simulink model "turbo_controller"  (R2025a)
settings: Solver=FixedStepAuto  StartTime=0.0  StopTime=inf  FixedStep=0.001  RelTol=1e-3
PostLoadFcn:
  | % 自动定位同目录CubeMX文件；不需要外部初始化脚本。
  | codertarget.data.setParameterValue('turbo_controller','STM32CubeMX.ProjectFile',fullfile(fileparts(get_param('turbo_controller','FileName')),'turbo_f407.ioc'));
InitFcn:
  | % 中文说明：按原控制器字段与类型创建三组接口总线；控制参数已内嵌。
  | tc_names=["EValve_Cycle" "EValve_Open" "Eblast_Cycle" "Eblast_Open" "Motor_Cycle" "Motor_Open" "EValve_Enable" "Eblast_Enable" "Motor_Enable" "SWO_Firework" "SWO_BleedAir" "EngineState" "Flag_ECUReset_Clear" "Flag_ECUReset_Save" "Flag_Reset_Enable" "Accelerator" "Nc_dem" "Nc"]; tc_types=["uint16" "uint16" "uint16" "uint16" "uint16" "uint16" "uint8" "uint8" "uint8" "uint8" "uint8" "uint8" "uint8" "uint8" "uint8" "single" "single" "single"];
  | for tc_k=1:numel(tc_names)
  |  tc_e(tc_k)=Simulink.BusElement; tc_e(tc_k).Name=char(tc_names(tc_k)); tc_e(tc_k).DataType=char(tc_types(tc_k));
  | end
  | EngineControl_Out=Simulink.Bus; EngineControl_Out.DataScope='Exported'; EngineControl_Out.Elements=tc_e;
  | clear tc_e tc_names tc_types tc_k
  | tc_names=["savedata1" "savedata2" "savedata3" "savedata4" "savedata5" "savedata6" "savedata7" "savedata8" "savedata9" "savedata10" "savedata11" "savedata12" "savedata13" "savedata14" "savedata15" "savedata16" "savedata17" "savedata18" "savedata19" "savedata20" "savedata21" "savedata22" "savedata23" "savedata24" "savedata25"]; tc_types=["single" "single" "single" "single" "single" "single" "single" "single" "single" "single" "single" "single" "single" "single" "single" "single" "single" "single" "single" "single" "single" "single" "single" "single" "single"];
  | for tc_k=1:numel(tc_names)
  |  tc_e(tc_k)=Simulink.BusElement; tc_e(tc_k).Name=char(tc_names(tc_k)); tc_e(tc_k).DataType=char(tc_types(tc_k));
  | end
  | SaveData_Out=Simulink.Bus; SaveData_Out.DataScope='Exported'; SaveData_Out.Elements=tc_e;
  | clear tc_e tc_names tc_types tc_k
  | tc_names=["senddata1" "senddata2" "senddata3" "senddata4" "senddata5" "senddata6" "senddata7" "senddata8" "senddata9" "senddata10" "senddata11" "senddata12" "senddata13" "senddata14" "senddata15" "senddata16" "senddata17" "senddata18" "senddata19" "senddata20" "senddata21" "senddata22" "senddata23" "senddata24" "senddata25" "senddata26" "senddata27" "senddata28" "senddata29"]; tc_types=["uint8" "uint8" "uint8" "uint8" "uint8" "uint8" "uint8" "uint8" "uint8" "uint8" "uint8" "uint8" "uint8" "uint8" "uint8" "uint8" "uint8" "uint8" "uint8" "uint8" "uint8" "uint8" "uint8" "uint8" "uint8" "uint8" "uint8" "uint8" "uint8"];
  | for tc_k=1:numel(tc_names)
  |  tc_e(tc_k)=Simulink.BusElement; tc_e(tc_k).Name=char(tc_names(tc_k)); tc_e(tc_k).DataType=char(tc_types(tc_k));
  | end
  | SendData_Out=Simulink.Bus; SendData_Out.DataScope='Exported'; SendData_Out.Elements=tc_e;
  | clear tc_e tc_names tc_types tc_k
  | 
  | % 以下为接口中文说明；只设置描述，不改变数值或数据类型。
  | EngineControl_Out.Description='执行控制输出（阀、电机、点火、状态及复位请求）';
  | tc_cn=["EValve_Cycle（主油阀周期计数（每计数2毫秒））" "EValve_Open（主油阀开通计数（每计数2毫秒））" "Eblast_Cycle（副油阀周期计数（每计数2毫秒））" "Eblast_Open（副油阀开通计数（每计数2毫秒））" "Motor_Cycle（起动电机周期计数）" "Motor_Open（起动电机开通计数）" "EValve_Enable（主油阀驱动使能）" "Eblast_Enable（副油阀驱动使能）" "Motor_Enable（起动电机使能）" "SWO_Firework（点火器使能（1开））" "SWO_BleedAir（引气阀使能（1开））" "EngineState（发动机状态）" "Flag_ECUReset_Clear（清除复位恢复状态请求）" "Flag_ECUReset_Save（保存复位恢复数据请求）" "Flag_Reset_Enable（处理器软件复位请求）" "Accelerator（油门／油泵给定控制量）" "Nc_dem（控制目标转速）" "Nc（发动机反馈转速（转每分））"];
  | tc_elements=EngineControl_Out.Elements;
  | for tc_k=1:numel(tc_cn)
  |  tc_elements(tc_k).Description=char(tc_cn(tc_k));
  | end
  | EngineControl_Out.Elements=tc_elements;
  | clear tc_cn tc_elements tc_k
  | SaveData_Out.Description='25项运行记录；字段含义按当前模型数据来源解释';
  | tc_cn=["savedata1（指令回显记录）" "savedata2（入口总温记录（℃））" "savedata3（电源电压记录）" "savedata4（排气温度记录（℃））" "savedata5（标定燃油压力记录）" "savedata6（副油阀占空比记录（％））" "savedata7（主油阀占空比记录（％））" "savedata8（温度修正转速记录）" "savedata9（开关输出及反馈位域）" "savedata10（物理转速记录）" "savedata11（油泵目标给定原始值）" "savedata12（起动电机占空比记录（％））" "savedata13（发动机状态码记录）" "savedata14（故障告警位域记录）" "savedata15（模型记录帧序号）" "savedata16（处理器温度记录（℃））" "savedata17（装订转速记录（沿用旧电源字段名））" "savedata18（导航高度记录）" "savedata19（飞行空速记录）" "savedata20（主阀旧记录位（恒零保留））" "savedata21（第21项保留记录（恒零））" "savedata22（保留记录项22）" "savedata23（保留记录项23）" "savedata24（保留记录项24）" "savedata25（保留记录项25）"];
  | tc_elements=SaveData_Out.Elements;
  | for tc_k=1:numel(tc_cn)
  |  tc_elements(tc_k).Description=char(tc_cn(tc_k));
  | end
  | SaveData_Out.Elements=tc_elements;
  | clear tc_cn tc_elements tc_k
  | SendData_Out.Description='29字段回传及外设命令接口；板端上位机帧只取第3至27字段';
  | tc_cn=["senddata1（回传发送允许标志（不直接上线路））" "senddata2（回传载荷长度25字节）" "senddata3（回传指令回显字节）" "senddata4（总温编码字节（℃＋80））" "senddata5（电源电压编码字节）" "senddata6（排温编码高字节）" "senddata7（排温编码低字节）" "senddata8（燃油压力编码高字节）" "senddata9（燃油压力编码低字节）" "senddata10（副油阀占空比字节（％））" "senddata11（主油阀占空比字节（％））" "senddata12（修正转速编码高字节）" "senddata13（修正转速编码低字节）" "senddata14（驱动及反馈状态位域）" "senddata15（物理转速编码高字节）" "senddata16（物理转速编码低字节）" "senddata17（油泵目标给定高字节（串口二使用））" "senddata18（油泵目标给定低字节（串口二使用））" "senddata19（起动电机占空比命令（串口一使用））" "senddata20（发动机状态码字节）" "senddata21（故障告警位域字节）" "senddata22（帧序号占位（板端另行填写））" "senddata23（处理器温度编码（℃＋50））" "senddata24（控制目标转速编码高字节）" "senddata25（控制目标转速编码低字节）" "senddata26（占位字节（板端改填实测泵速高字节））" "senddata27（占位字节（板端改填实测泵速低字节））" "senddata28（装订转速高字节（本板未发送））" "senddata29（装订转速低字节（本板未发送））"];
  | tc_elements=SendData_Out.Elements;
  | for tc_k=1:numel(tc_cn)
  |  tc_elements(tc_k).Description=char(tc_cn(tc_k));
  | end
  | SendData_Out.Elements=tc_elements;
  | clear tc_cn tc_elements tc_k
  | 
  | 
  | % FRAM模块化事务：接口类型和上电初始状态，随模型保存，无外部初始化文件。
  | clear FM_elements
  | FM_elements(1)=Simulink.BusElement;FM_elements(1).Name='phase';FM_elements(1).DataType='uint8';FM_elements(1).Dimensions=[1 1];FM_elements(1).Description='phase（当前事务阶段）';
  | FM_elements(2)=Simulink.BusElement;FM_elements(2).Name='a';FM_elements(2).DataType='uint8';FM_elements(2).Dimensions=[64 1];FM_elements(2).Description='a（启动时缓存的首区64字节）';
  | FM_elements(3)=Simulink.BusElement;FM_elements(3).Name='active';FM_elements(3).DataType='uint16';FM_elements(3).Dimensions=[1 1];FM_elements(3).Description='active（当前有效记录区地址）';
  | FM_elements(4)=Simulink.BusElement;FM_elements(4).Name='generation';FM_elements(4).DataType='uint32';FM_elements(4).Dimensions=[1 1];FM_elements(4).Description='generation（当前有效记录代号）';
  | FM_elements(5)=Simulink.BusElement;FM_elements(5).Name='record';FM_elements(5).DataType='uint8';FM_elements(5).Dimensions=[64 1];FM_elements(5).Description='record（本次冻结的待写记录）';
  | FM_elements(6)=Simulink.BusElement;FM_elements(6).Name='addr';FM_elements(6).DataType='uint16';FM_elements(6).Dimensions=[1 1];FM_elements(6).Description='addr（本次备用写入地址）';
  | FM_elements(7)=Simulink.BusElement;FM_elements(7).Name='lastSave';FM_elements(7).DataType='single';FM_elements(7).Dimensions=[1 1];FM_elements(7).Description='lastSave（上次开始保存的秒数）';
  | FM_elements(8)=Simulink.BusElement;FM_elements(8).Name='lastState';FM_elements(8).DataType='uint8';FM_elements(8).Dimensions=[1 1];FM_elements(8).Description='lastState（上次保存时的发动机状态）';
  | FM_elements(9)=Simulink.BusElement;FM_elements(9).Name='boot';FM_elements(9).DataType='boolean';FM_elements(9).Dimensions=[1 1];FM_elements(9).Description='boot（启动记录是否允许恢复）';
  | FM_elements(10)=Simulink.BusElement;FM_elements(10).Name='consumed';FM_elements(10).DataType='boolean';FM_elements(10).Dimensions=[1 1];FM_elements(10).Description='consumed（本次启动恢复通知是否已发送）';
  | FM_elements(11)=Simulink.BusElement;FM_elements(11).Name='payload';FM_elements(11).DataType='uint8';FM_elements(11).Dimensions=[20 1];FM_elements(11).Description='payload（当前20字节恢复内容）';
  | ... (+35 lines)
model workspace (MAT data in the model file):
  CRC16_Table_Reference = [0 4129 8258 12387 16516 20645 24774 28903 33032 37161 41290 45419 ... (256 elements, 256x1)]
  PE_Kaer = [0.15402 0.15402 0.12264 0.10076 0.09481 0.07601 0.07111 0.0569 0.05198 0.04926 0.05308 0.04325 ... (13 elements, 1x13)]
  PE_Nr = [21.2982 61.4260372 67.7475458 72.7394382 76.845934 80.6988798 83.8449282 86.6491912 88.9382406 89.178606 91.1938214 93.4068058 ... (13 elements, 1x13)]
  PE_Pump_Translate = 33.5999984741
  PE_RotaSpeed_Translate = 860
  PE_Taer = [0.4939154 0.4939154 0.40780982 0.34066978 0.31622756 0.30405716 0.34300244 0.26785022 0.37393554 0.23914836 0.44563948 0.31044662 ... (13 elements, 1x13)]
  PF_ACCFULLRANGE = 3360
  PF_Flag_ECUReset = 0
  PF_Flag_rx_suc = 1
  PF_Gear_Info = [40000; 45000; 50000; 55000; 57000; 59000; 60000; 61000; 61000; 61000; 61000; 61000]
  PF_K_TiaoJie = 1
  PF_Kpu = 10
  PF_MySet_Rxdata = [0 0 0 0 0 0 0 0 0 0 0 0 ... (50 elements, 50x1)]
  PF_MyUsart1_Rxdata = [0 0 0 0 0 0 0 0 0 0 0 0 ... (50 elements, 50x1)]
  PF_MyUsart2_Rxdata = [0 0 0 0 0 0 0 0 0 0 0 0 ... (50 elements, 50x1)]
  PF_Reset_Information = [0 0 0 0 0 0 0 0 0 0 0 0 ... (20 elements, 20x1)]
  PF_Sensor_X1_T4 = [0 4095]
  PF_Sensor_X2_T4 = [0 1.66666698456]
  PF_Sensor_X3_T4 = [0 504 999 1497 2010 2529 3051 3568 4076 4571 4959]
  PF_Sensor_X_P2 = [0.5 3]
  PF_Sensor_X_Poil = [0.5 3]
  PF_Sensor_X_T1t = [-50 300]
  PF_Sensor_X_Vpower = [0 3]
  PF_Sensor_X_Vpump = [0 3]
  PF_Sensor_Y1_T4 = [0 3]
  PF_Sensor_Y2_T4 = [0 5000]
  PF_Sensor_Y3_T4 = [0 100 200 300 400 500 600 700 800 900 980]
  PF_Sensor_Y_P2 = [0 1000]
  PF_Sensor_Y_Poil = [0 1000]
  PF_Sensor_Y_T1t = [-50 300]
  PF_Sensor_Y_Vpower = [0 33]
  PF_Sensor_Y_Vpump = [0 33]
  PG_CtrlMode_CloseLoop : mpt.Parameter (value not decoded)
  PG_CtrlMode_ManualAcc : mpt.Parameter (value not decoded)
  PG_CtrlMode_Origin : mpt.Parameter (value not decoded)
  PG_CtrlMode_Start : mpt.Parameter (value not decoded)
  PG_CtrlMode_Stop : mpt.Parameter (value not decoded)
  PG_ES_Clp : mpt.Parameter (value not decoded)
  PG_ES_EngStart : mpt.Parameter (value not decoded)
  PG_ES_Manual : mpt.Parameter (value not decoded)
  PG_ES_Origin : mpt.Parameter (value not decoded)
  PG_ES_Stop : mpt.Parameter (value not decoded)
  PG_Instr_BleedAirSet : mpt.Parameter (value not decoded)
  PG_Instr_CloseLoop : mpt.Parameter (value not decoded)
  PG_Instr_ECUReSet : mpt.Parameter (value not decoded)
  PG_Instr_EValveSet : mpt.Parameter (value not decoded)
  PG_Instr_EblastSet : mpt.Parameter (value not decoded)
  PG_Instr_Erase : mpt.Parameter (value not decoded)
  PG_Instr_FireWorkSet : mpt.Parameter (value not decoded)
  PG_Instr_ManualPlus : mpt.Parameter (value not decoded)
  PG_Instr_ManualrReduce : mpt.Parameter (value not decoded)
  PG_Instr_MotorSet : mpt.Parameter (value not decoded)
  PG_Instr_OilSet : mpt.Parameter (value not decoded)
  PG_Instr_SelfCheck : mpt.Parameter (value not decoded)
  PG_Instr_Start : mpt.Parameter (value not decoded)
  PG_Instr_Stop : mpt.Parameter (value not decoded)
  PG_Instr_StopZero : Simulink.Parameter (value not decoded)
  PG_Location_Air : Simulink.Parameter (value not decoded)
  PG_Location_Gnd : Simulink.Parameter (value not decoded)
  PG_ServoCtrlMode_CloseLoop : Simulink.Parameter (value not decoded)
  PG_ServoCtrlMode_CloseLoopMax : Simulink.Parameter (value not decoded)
  PG_ServoCtrlMode_CloseLoopMin : Simulink.Parameter (value not decoded)
  PG_ServoCtrlMode_ManualAcc : Simulink.Parameter (value not decoded)
  PG_ServoCtrlMode_ManualAccMax : Simulink.Parameter (value not decoded)
  PG_ServoCtrlMode_ManualAccMin : Simulink.Parameter (value not decoded)
  PG_SpeedDot_Permit : Simulink.Parameter (value not decoded)
  PL_EngineModel_Actuator = [0 10 100]
  PL_EngineModel_EngineStar_Press_P2 = [1013 1098.4 1099.144828 1099.931034 1103.613793 1162.662069 1143.793103 1131.006897 1123.186207 1117.6 1114 1111.806897 ... (127 elements, 1x127)]
  PL_EngineModel_EngineStar_RotaSpeed = [200 2000 9584 9660 10220 10240 10260 10288 10308 10368 10380 10408 ... (127 elements, 1x127)]
  PL_EngineModel_EngineStar_Temp_Exhaust = [128 129 129.1 130 131 131.1 132 133 134 134.1 135 135.1 ... (127 elements, 1x127)]
  PL_EngineModel_EngineStar_Time = [0.05 0.1 0.15 0.2 0.25 0.3 0.35 0.4 0.45 0.5 0.55 0.6 ... (127 elements, 1x127)]
  PL_EngineModel_IdleAbove_Nr = [0 21.2982 61.4260372 67.7475458 72.7394382 76.845934 80.6988798 83.8449282 86.6491912 88.9382406 89.178606 91.1938214 ... (14 elements, 1x14)]
  PL_EngineModel_IdleAbove_P2r = [0.986923266716 1.57907722675 1.81593881076 1.99358499877 2.23044658278 2.43770046879 2.65482358747 2.84233900814 3.03972366149 3.18776215149 3.25684678016 3.3950160375 ... (14 elements, 1x14)]
  PL_EngineModel_IdleAbove_Tempr = [0.0536001429337 1.07200285867 1.63301768805 1.63659103091 1.66875111667 1.72592460247 1.77595140254 1.86171163123 1.95461854565 2.03323208862 2.03323208862 2.13685903162 ... (14 elements, 1x14)]
  PL_EngineModel_IdleAbove_Ter = [0.42434128 0.42434128 0.42434128 0.30669408 0.23570008 0.22150128 0.1997974 0.23803274 0.16115638 0.24279948 0.13600422 0.31308354 ... (14 elements, 1x14)]
  PL_EngineModel_IdleAbove_Wfr = [0 10.142 23.8337 27.8905 31.9473 36.0041 40.0609 44.1177 48.1745 52.2313 52.7384 56.7952 ... (14 elements, 1x14)]
  PL_EngineModel_Press_P2 = [400 400 400 400 400 400 400 400 400 400]
  PL_EngineModel_Rotaspeed = [0 20000 96400]
  PL_EngineModel_Temp_Exhaust = [500 500 500 500 500 500 500 500 500 500]
  PL_Kaer = [0.1 0.1 0.1 0.1 0.1 0.1]
  PL_Nr = [50 60 70 80 90 100]
  PL_Taer = [0.1 0.1 0.1 0.1 0.1 0.1]
  Sig : Simulink.Signal (value not decoded)
  Ts_ms : Simulink.Parameter (value not decoded)
  false : Simulink.Parameter (value not decoded)
  true : Simulink.Parameter (value not decoded)
symbols that are objects in the model workspace (value not decoded): PG_CtrlMode_CloseLoop, PG_CtrlMode_ManualAcc, PG_CtrlMode_Origin, PG_CtrlMode_Start, PG_CtrlMode_Stop, PG_ES_Clp, PG_ES_EngStart, PG_ES_Manual, PG_ES_Origin, PG_ES_Stop, PG_Instr_BleedAirSet, PG_Instr_CloseLoop, PG_Instr_EblastSet, PG_Instr_ECUReSet, PG_Instr_Erase, PG_Instr_EValveSet, PG_Instr_FireWorkSet, PG_Instr_ManualPlus, PG_Instr_ManualrReduce, PG_Instr_MotorSet, PG_Instr_OilSet, PG_Instr_SelfCheck, PG_Instr_Start, PG_Instr_Stop, PG_Instr_StopZero, PG_ServoCtrlMode_CloseLoop, PG_ServoCtrlMode_CloseLoopMax, PG_ServoCtrlMode_CloseLoopMin, PG_ServoCtrlMode_ManualAcc, PG_ServoCtrlMode_ManualAccMax, PG_ServoCtrlMode_ManualAccMin, Ts_ms
libraries: simulink x97, stm32blockslib x10, stm32f4xxblockslib x8
(part 8 of 26)

== system turbo_controller/BoardOutput_串口封装与阀门时序/Out04_Command（电机及油泵指令） ==
  note: 给电机和油泵各生成一帧控制命令
      |
      | 这里使用上层执行控制和回传字段，按20 ms节拍生成两路外设命令，而不是解析外设回包。两路协议
      | 均为9字节：
      | AA 55 03 00 02 命令高字节 命令低字节 CRC高字节 CRC低字节。
      |
      | 电机这一路把命令高字节固定为0，低字节采用原电机给定。油泵这一路采用原有油泵给定的高低两个
      | 字节；不能把两路的字节来源互换。
      | MotorFrame和PumpFrame各自只对两个命令字节计算CRC，不把前五项固定头部加入校验。
      |
      | 到20 ms更新且相应发送条件成立时，输出帧和有效长度交Out05_Handoff，再送根层USART1/USART2发
      | 送模块。数据值为0也可能是一条有意义的停机命令，因此发送许可和命令是否为0是不同判断。
  Send（外设命令总线）_867 : Inport  OutDataTypeStr=Bus: SendData_Out
  Seconds（当前秒数）_868 : Inport  Port=2  OutDataTypeStr=double
  Commands（原油泵与电机给定字节）_876 : BusSelector  OutputSignals=senddata17,senddata18,senddata19
  Constant（常量）_869 : Constant  Value=1000  OutDataTypeStr=double
  Constant（常量）_872 : Constant  Value=20  OutDataTypeStr=double
  Constant（常量）_874 : Constant  Value=0  OutDataTypeStr=double
  Constant（常量）_924 : Constant  Value=0  OutDataTypeStr=uint8
  Constant（常量）_975 : Constant  Value=9  OutDataTypeStr=uint16
  Constant（常量）_976 : Constant  Value=0  OutDataTypeStr=uint16
  Every20ms（20毫秒更新许可）_875 : RelationalOperator  Operator===  OutDataTypeStr=boolean  RndMeth=Simplest  InputSameDT=off
  Format（保持原输出维度）_2 : Reshape
  Format（保持原输出维度）_4 : Reshape
  Length（二十毫秒发送九字节）_977 : Switch  Criteria=u2 ~= 0  SaturateOnIntegerOverflow=off  InputSameDT=off
  Milliseconds（秒换算为毫秒）_870 : Product  Inputs=**  SaturateOnIntegerOverflow=on  OutDataTypeStr=Inherit: Same as first input
  MotorFrame（电机指令高字节固定为零）_925 : Subsystem  Description=|
      | 电机的两个命令字节怎样装成九字节帧
      | 
      | 父级把高命令字节固定0，低命令字节来自电机给定。这里不重新决定给定大小，只把这两个字节包装为外设协议。
      | 
      | 前五项固定为十六进制AA、55、03、00、02；第6、7项依次放命令高字节与低字节。CRC16只以第6、7两项为输入，计算出16位校验值，再把CRC高字节放第8项、低字节放第9项。
      | 
      | 完整帧 = [AA;55;03;00;02;CmdH;CmdL;CRCH;CRCL]。
      | 例如命令高0、低100表示两字节数100；CRC必须用[0,100]按本工程CRC表算出，不能只校验100或把AA55头部也算进去。
      | 
      | 9项帧交给父级，由20 ms发送许可和长度控制是否实际发送；本模块本身不操作串口。
  NoFrame（非通信毫秒输出零帧）_974 : Constant  Value=zeros(9,1)  OutDataTypeStr=uint8
  Phase20（20毫秒相位）_873 : Math  Operator=mod
  PumpFrame（油泵指令使用原高低给定字节）_973 : Subsystem  Description=|
      | 油泵的两个命令字节怎样装成九字节帧
      | 
      | 父级传入原油泵给定的高、低两个命令字节。这里不重新决定给定大小，只把这两个字节包装为外设协议。
      | 
      | 前五项固定为十六进制AA、55、03、00、02；第6、7项依次放命令高字节与低字节。CRC16只以第6、7两项为输入，计算出16位校验值，再把CRC高字节放第8项、低字节放第9项。
      | 
      | 完整帧 = [AA;55;03;00;02;CmdH;CmdL;CRCH;CRCL]。
      | 例如命令高0、低100表示两字节数100；CRC必须用[0,100]按本工程CRC表算出，不能只校验100或把AA55头部也算进去。
      | 
      | 9项帧交给父级，由20 ms发送许可和长度控制是否实际发送；本模块本身不操作串口。
  RoundTime（按原规则取整）_871 : Rounding  Operator=round
  Select（按条件选择）_978 : Switch  Criteria=u2 ~= 0  SaturateOnIntegerOverflow=off  InputSameDT=off
  Select（按条件选择）_982 : Switch  Criteria=u2 ~= 0  SaturateOnIntegerOverflow=off  InputSameDT=off
  Tx1（电机九字节指令）_979 : Reshape  OutputDimensionality=Column vector (2-D)
  Tx2（油泵九字节指令）_983 : Reshape  OutputDimensionality=Column vector (2-D)
  Tx1（电机九字节指令）_980 : Outport
  Length1（电机发送长度）_981 : Outport  Port=2
  Tx2（油泵九字节指令）_984 : Outport  Port=3
  Length2（油泵发送长度）_985 : Outport  Port=4
  wires:
  Tx2（油泵九字节指令）_983/1 -> Tx2（油泵九字节指令）_984/1  "Tx2（油泵九字节指令）"
  Select（按条件选择）_982/1 -> Tx2（油泵九字节指令）_983/1  "Select（按条件选择）"
  PumpFrame（油泵指令使用原高低给定字节）_973/1(Frame（含校验的完整指令帧）_972) -> Select（按条件选择）_982/1  "PumpFrame（油泵指令使用原高低给定字节）"
  Tx1（电机九字节指令）_979/1 -> Tx1（电机九字节指令）_980/1  "Tx1（电机九字节指令）"
  Select（按条件选择）_978/1 -> Tx1（电机九字节指令）_979/1  "Select（按条件选择）"
  NoFrame（非通信毫秒输出零帧）_974/1 -> Select（按条件选择）_982/3, Select（按条件选择）_978/3  "NoFrame（非通信毫秒输出零帧）"
  MotorFrame（电机指令高字节固定为零）_925/1(Frame（含校验的完整指令帧）_923) -> Select（按条件选择）_978/1  "MotorFrame（电机指令高字节固定为零）"
  Commands（原油泵与电机给定字节）_876/2 -> PumpFrame（油泵指令使用原高低给定字节）_973/2(LowByte（给定低字节）_928)  "<senddata18>"
  Commands（原油泵与电机给定字节）_876/1 -> PumpFrame（油泵指令使用原高低给定字节）_973/1(HighByte（给定高字节）_926)  "<senddata17>"
  Commands（原油泵与电机给定字节）_876/3 -> MotorFrame（电机指令高字节固定为零）_925/2(LowByte（给定低字节）_879)  "<senddata19>"
  Constant（常量）_924/1 -> MotorFrame（电机指令高字节固定为零）_925/1(HighByte（给定高字节）_877)  "Constant（常量）"
  Send（外设命令总线）_867/1 -> Commands（原油泵与电机给定字节）_876/1  "Send（外设命令总线）"
  Constant（常量）_874/1 -> Every20ms（20毫秒更新许可）_875/2  "Constant（常量）"
  Phase20（20毫秒相位）_873/1 -> Every20ms（20毫秒更新许可）_875/1  "Phase20（20毫秒相位）"
  Constant（常量）_872/1 -> Phase20（20毫秒相位）_873/2  "Constant（常量）"
  RoundTime（按原规则取整）_871/1 -> Phase20（20毫秒相位）_873/1  "RoundTime（按原规则取整）"
  Milliseconds（秒换算为毫秒）_870/1 -> RoundTime（按原规则取整）_871/1  "Milliseconds（秒换算为毫秒）"
  Constant（常量）_869/1 -> Milliseconds（秒换算为毫秒）_870/2  "Constant（常量）"
  Seconds（当前秒数）_868/1 -> Milliseconds（秒换算为毫秒）_870/1  "Seconds（当前秒数）"
  Format（保持原输出维度）_4/1 -> Length2（油泵发送长度）_985/1
  Format（保持原输出维度）_2/1 -> Length1（电机发送长度）_981/1
  Constant（常量）_975/1 -> Length（二十毫秒发送九字节）_977/1  "Constant（常量）"
  Every20ms（20毫秒更新许可）_875/1 -> Select（按条件选择）_982/2, Length（二十毫秒发送九字节）_977/2, Select（按条件选择）_978/2  "Every20ms（20毫秒更新许可）"
  Constant（常量）_976/1 -> Length（二十毫秒发送九字节）_977/3  "Constant（常量）"
  Length（二十毫秒发送九字节）_977/1 -> Format（保持原输出维度）_2/1, Format（保持原输出维度）_4/1  "Length（二十毫秒发送九字节）"

== system turbo_controller/BoardOutput_串口封装与阀门时序/Out05_Handoff（输出交接与软件复位） ==
  note: 把准备好的输出交给硬件并处理复位请求
      |
      | 上游已经完成电平时序、上位机帧、电机帧和油泵帧。本层把这些结果按固定字段组成交接总线，转回
      | 根层GPIO与UART模块所需的端口，不在这里重新计算温压或改变控制模式。
      |
      | 串口的数据数组和有效长度必须配套：长度为0表示本周期不发送，命令内容为0却可能是有效的停泵/
      | 停电机帧，不能据数值0丢弃。
      |
      | 另一支取出Flag_Reset_Enable，与0比较后转成复位服务的0/1执行许可。ResetService只在请求有效
      | 时执行目标端软件复位；正常电脑仿真走空实现。
      |
      | 输入依赖使复位处理与本周期输出计算有明确交接关系，但它没有等待硬件UART发送完成的反馈。因此
      | 不能把这里解释为已经确认所有字节发完才复位。
  Control（执行控制总线）_986 : Inport  OutDataTypeStr=Bus: EngineControl_Out
  portE（E口三路电平）_987 : Inport  Port=2
  portD（D口三路电平）_988 : Inport  Port=3
  tx4（上位机回传帧）_989 : Inport  Port=4
  len4（上位机回传长度）_990 : Inport  Port=5
  tx1（电机指令帧）_991 : Inport  Port=6
  len1（电机发送长度）_992 : Inport  Port=7
  tx2（油泵指令帧）_993 : Inport  Port=8
  len2（油泵发送长度）_994 : Inport  Port=9
  BoardOutputs（按原字段顺序统一输出）_995 : BusCreator  Inputs=8  OutDataTypeStr=Bus: BO_Output  NonVirtualBus=on
      settings: InheritFromInputs=off
  Constant（常量）_998 : Constant  Value=0  OutDataTypeStr=uint8
  ResetCount（请求换算为零次或一次） : DataTypeConversion  OutDataTypeStr=uint32  SaturateOnIntegerOverflow=off  RndMeth=Floor
  ResetFlag（读取允许软件复位标志）_997 : BusSelector  OutputSignals=Flag_Reset_Enable
  ResetRequested（复位标志非零）_999 : RelationalOperator  Operator=~=  OutDataTypeStr=boolean  RndMeth=Simplest  InputSameDT=off
  ResetService（ST官方软件复位服务） : Subsystem  Description=|  Priority=100  TreatAsAtomicUnit=on
      | 什么时候调用STM32软件复位
      | 
      | 父级把非零复位请求转换成0或1次执行许可。这里用这个次数决定本次是否进入ExecutionMode：0次完全不调用，1次才执行对应运行方式的实现。
      | 
      | 普通计算机仿真采用Simulation分支，该分支为空，不尝试复位电脑。生成目标代码采用Target分支，用官方C Caller调用CMSIS的NVIC_SystemReset，让STM32重新进入启动流程。
      | 
      | 这里不是清零一个控制变量，而是最终硬件复位服务。要保存运行状态，应在复位前由上层FRAM事务完成对应保存；本模块不负责CRC、写入验证或恢复记录选择。
  Output（完整板级输出总线）_996 : Outport
  wires:
  Constant（常量）_998/1 -> ResetRequested（复位标志非零）_999/2  "Constant（常量）"
  ResetFlag（读取允许软件复位标志）_997/1 -> ResetRequested（复位标志非零）_999/1  "<Flag_Reset_Enable>"
  Control（执行控制总线）_986/1 -> ResetFlag（读取允许软件复位标志）_997/1  "Control（执行控制总线）"
  BoardOutputs（按原字段顺序统一输出）_995/1 -> Output（完整板级输出总线）_996/1  "BoardOutputs（按原字段顺序统一输出）"
  len2（油泵发送长度）_994/1 -> BoardOutputs（按原字段顺序统一输出）_995/8  "len2（油泵发送长度）"
  tx2（油泵指令帧）_993/1 -> BoardOutputs（按原字段顺序统一输出）_995/7  "tx2（油泵指令帧）"
  len1（电机发送长度）_992/1 -> BoardOutputs（按原字段顺序统一输出）_995/6  "len1（电机发送长度）"
  tx1（电机指令帧）_991/1 -> BoardOutputs（按原字段顺序统一输出）_995/5  "tx1（电机指令帧）"
  len4（上位机回传长度）_990/1 -> BoardOutputs（按原字段顺序统一输出）_995/4  "len4（上位机回传长度）"
  tx4（上位机回传帧）_989/1 -> BoardOutputs（按原字段顺序统一输出）_995/3  "tx4（上位机回传帧）"
  portD（D口三路电平）_988/1 -> BoardOutputs（按原字段顺序统一输出）_995/2  "portD（D口三路电平）"
  portE（E口三路电平）_987/1 -> BoardOutputs（按原字段顺序统一输出）_995/1  "portE（E口三路电平）"
  ResetCount（请求换算为零次或一次）/1 -> ResetService（ST官方软件复位服务）/1(Request（复位请求零或一）_1545)
  ResetRequested（复位标志非零）_999/1 -> ResetCount（请求换算为零次或一次）/1  "ResetRequested（复位标志非零）"

== system turbo_controller/CLM/ClpControl ==
  note: 闭环怎样根据转速偏差调整油泵
      |
      | 本模块在发动机闭环模式运行。输入S_SPM含目标转速、实际滤波转速和入口压力，S_FAM提供转速故障
      | 标志，上一执行总线提供上次油泵给定。这里的Accelerator是油泵给定控制量，不能直接当作角度或
      | 占空比。
      |
      | 先由Aim__Parameter_Calculate限制目标变化、给出油泵上下限和Kp/Ki。目标进入闭环时从当前转速
      | 逐步移动，避免突然把一个远离实际值的装订量全部加到控制律。
      | CtrlLaw计算目标减反馈的误差，用增量PI算本周期油泵变化量；小误差保持旧值，变化量按入口压力
      | 缩放并限幅。
      |
      | Fault_Process再看转速传感器故障：短时故障可冻结上次给定，锁存故障时改用装订转速/高度插值的
      | 备用给定，并限制变化步长。正常时采用PI结果。
      | 最终候选给定和Kp/Ki、目标、给定上下限等参数组成闭环输出总线，交ControlOut_Manage再做模式统
      | 一选择；不会直接在这里发送油泵串口命令。
  note: DaYu5000
      | DaYu5000：只判断一个条件
      |
      | 把输入与5000比较，使用关系“>=”。成立输出1，不成立输出0；输出是判断标志，不是把输入缩放成
      | 该常数。
      |
      | 比较门限用于父级的分支条件，没有滤波、延时确认或锁存。例如输入恰好等于门限时，“>=、<=、==
      | ”成立，“>、<”不成立。是否需要持续确认或同时满足其他条件，由父级连线决定。
  S_SPM : Inport
      settings: AttributesFormatString=S_SPM（通信及传感器信息总线）
  S_FAM : Inport  Port=2
      settings: AttributesFormatString=S_FAM（故障标志总线）
  S_ServoOut_Last : Inport  Port=3
      settings: AttributesFormatString=S_ServoOut_Last（伺服输出上一周期）
  Action Port : ActionPort  InitializeStates=reset  ActionPortLabel=case [ 2 ]:
      settings: AttributesFormatString=Action Port（动作端口）
  Aim__Parameter_Calculate : Subsystem  Description=|
      | 闭环计算之前要准备哪些参数
      | 
      | 本层把反馈转速和上位机装订需求整理成一套控制参数，供CtrlLaw直接使用，不在这里计算最终油泵给定。
      | 
      | Aim_AccMaxMin_Cal1先用进入闭环时的反馈值作为起点，对装订需求作上升/下降限制，得到目标Nc_dem；目标不低于40000，当前给定下限为700、上限为8000。
      | PIParameter_Cal分别按实际转速与目标转速查表，获得两套Kp/Ki候选，再各取较小值作为本次系数。允许转速误差固定为300。
      | 
      | 结果按字段打包为允许误差、目标转速、油泵下限、油泵上限、Kp、Ki六项。例如装订从40000升到50000，实际控制目标不会直接跳50000，而先经HoldFirst逐次逼近；系数也随目标/反馈工作点变化。
      | 
      | 这些字段送同级CtrlLaw和Fault_Process。总线打包只是交接参数，不能把它理解成又积分一次或又滤波一次。
      settings: AttributesFormatString=Aim__Parameter_Calculate（目标参数计算）
  Bus Creator : BusCreator  Inputs=9
      settings: AttributesFormatString=Bus Creator（总线创建器）
  Bus Selector : BusSelector  OutputSignals=Sensor（传感器信息总线）.Nc_Filter（滤波后转速）,COMM（通信信息总线）.SpeedLoad（装订转速）
      settings: AttributesFormatString=Bus Selector（总线选择器）
  Bus Selector1 : BusSelector  OutputSignals=RotaSpeed_ErrorAllow（转速允许偏差）,Kp（比例增益）,Ki（积分增益）,Nc_dem（控制目标转速）,Acc_Min（油泵给定下限）,Acc_Max（油泵给定上限）
      settings: AttributesFormatString=Bus Selector1（总线选择器1）
  Bus Selector2 : BusSelector  OutputSignals=Accelerator（油泵给定控制量）
      settings: AttributesFormatString=Bus Selector2（总线选择器2）
  CtrlLaw : Subsystem  Description=|
      | 增量PI怎样把转速偏差变成油泵给定
      | 
      | 输入包含当前目标、实际滤波转速、允许误差、Kp/Ki，以及上一周期油泵给定u_last。先求本次误差e=目标-反馈，Time Delay8保存上次误差e_prev。
      | 
      | 原始增量为：
      | Δu_raw=PF_K_TiaoJie×[Kp×(e-e_prev)+Ki×e]；
      | 当前PF_K_TiaoJie为1。Kp看误差变化，Ki看本次误差。这里已经是离散增量形式，不能再凭名称额外乘一次采样时间。
      | 
      | 入口总压先限在30～100，再除100得到q。增量限制在-10q～+10q之间，压力低时允许步长也变小。
      | 若abs(e)小于允许值300，输出直接保持u_last；否则输出u_last+限幅后的Δu。另一路S_Step_Acclerator输出这次限幅增量供记录/参数使用。
      | 
      | 例如q=1、计算增量为25，实际只加10；误差已在300以内时，即使算出小增量也采用保持支路。
      | 结果随后仍经过Fault_Process和模式仲裁，不能把本层候选给定当作已发送到油泵的最终命令。
      settings: AttributesFormatString=CtrlLaw（控制规律）
  DaYu5000 : simulink/Logic and Bit Operations/Compare To Constant  Description=|  relop=>=  const=5000  OutDataTypeStr=boolean
      | DaYu5000：只判断一个条件
      | 
      | 把输入与5000比较，使用关系“>=”。成立输出1，不成立输出0；输出是判断标志，不是把输入缩放成该常数。
      | 
      | 比较门限用于父级的分支条件，没有滤波、延时确认或锁存。例如输入恰好等于门限时，“>=、<=、==”成立，“>、<”不成立。是否需要持续确认或同时满足其他条件，由父级连线决定。
      settings: AttributesFormatString=DaYu5000（大于五千）
  Fault_Process : Subsystem  Description=|
      | 转速故障时油泵给定怎样切换
      | 
      | 本模块有正常PI候选值、上一周期油泵给定、转速故障Flag_NcFailure和锁存标志Lock_NcFailure，以及装订转速和高度。
      | 正常没有故障时，采用CtrlLaw的PI结果。
      | 
      | Flag_NcFailure成立但尚未锁存时，先保持上次给定，避免可疑转速让PI继续乱调。Lock_NcFailure成立时，改用D9-Nr-T5r生成的备用给定，优先级高于前面的普通保持选择。
      | 
      | 备用给定用装订转速和高度插值。三条高度曲线分别在40000与62000间给出对应给定：[2028,7342]、[1317,4148]、[702,1929]。高度先从m除1000转成km。结果再经GeneralFilter限到传入上下限，并按每次10的步长接近旧给定。
      | 
      | 因此故障锁存后不是凭空把油泵清零，而是走预设的备用控制曲线。最终仍交ControlOut_Manage按控制模式与边界统一仲裁。
      settings: AttributesFormatString=Fault_Process（故障处理）
  Gain{,1..5} (6 alike) : Gain
      Gain settings: AttributesFormatString=Gain（乘以系数1）
      Gain1 settings: AttributesFormatString=Gain1（乘以系数1）
      Gain2 settings: AttributesFormatString=Gain2（乘以系数1）
      Gain3 settings: AttributesFormatString=Gain3（乘以系数1）
      Gain4 settings: AttributesFormatString=Gain4（乘以系数1）
      Gain5 settings: AttributesFormatString=Gain5（乘以系数1）
  N1r_idle6 : Constant  Value=PG_CtrlMode_CloseLoop  OutDataTypeStr=uint8  SampleTime=-1
      settings: AttributesFormatString=N1r_idle6（一级转速归一化值慢车6）
  Scope1 : Scope
      settings: AttributesFormatString=Scope1（示波器1）  ActiveDisplayYMinimum=-57.5  ActiveDisplayYMaximum=817.5
  Signal Conversion : SignalConversion  OverrideOpt=off
      settings: AttributesFormatString=Signal Conversion（信号转换）
  Switch : Switch  Criteria=u2 ~= 0  SaturateOnIntegerOverflow=off  InputSameDT=off
      settings: AttributesFormatString=Switch（开关选择）
  dth = T0-288.1 : Constant  Value=0  OutDataTypeStr=uint8  SampleTime=-1
      settings: AttributesFormatString=dth = T0-288.1（固定常量0（旧名称不参与计算））
  dth = T0-288.6 : Constant  OutDataTypeStr=uint8  SampleTime=-1
      settings: AttributesFormatString=dth = T0-288.6（固定常量1（旧名称不参与计算））
  S_CtrlMode_CloseLoop : Outport  InitialOutput=[0]
      settings: AttributesFormatString=S_CtrlMode_CloseLoop（控制模式闭合回路）
  S_CloseLoop : Outport  Port=2  OutputWhenDisabled=reset  InitialOutput=[0]
      settings: AttributesFormatString=S_CloseLoop（闭合回路）
  wires:
  N1r_idle6/1 -> S_CtrlMode_CloseLoop/1
  S_SPM/1 -> [S_SPM], CtrlLaw/7(SPM), Bus Selector/1
  S_ServoOut_Last/1 -> Bus Selector2/1
  Aim__Parameter_Calculate/1(S_Control_Parameter) -> Bus Selector1/1
  Bus Selector1/5 -> Gain/1  "<Acc_Min（油泵给定下限）>"
  Bus Selector1/6 -> Gain1/1  "<Acc_Max（油泵给定上限）>"
  Bus Selector/1 -> [Nc_Filter], Aim__Parameter_Calculate/1(S_Nc_Filter)  "<Nc_Filter（滤波后转速）>"
  [Nc_Filter] -> CtrlLaw/6(S_Nc_Filter)
  S_FAM/1 -> Fault_Process/1(S_FAM)
  Bus Selector1/1 -> Gain5/1, CtrlLaw/2(S_RotaSpeed_ErrorAllow)  "<RotaSpeed_ErrorAllow（转速允许偏差）>"
  Bus Selector1/2 -> CtrlLaw/3(S_Kp), Gain4/1  "<Kp（比例增益）>"
  Bus Selector1/3 -> Gain3/1, CtrlLaw/4(S_Ki)  "<Ki（积分增益）>"
  Bus Selector1/4 -> Gain2/1, CtrlLaw/5(S_Nc_dem)  "<Nc_dem（控制目标转速）>"
  Bus Selector/2 -> Aim__Parameter_Calculate/2(S_Dem_SpeedLoad)  "<SpeedLoad（装订转速）>"
  Bus Creator/1 -> Signal Conversion/1
  CtrlLaw/2(S_Step_Acclerator) -> Bus Creator/2  "Step_Acclerator（阶跃油泵给定）"
  Signal Conversion/1 -> S_CloseLoop/1
  Gain/1 -> Fault_Process/5(Acc_Min), Bus Creator/3  "Close  LoopMin（闭环油泵给定下限）"
  Gain1/1 -> Fault_Process/6(Acc_Max), Bus Creator/4  "CloseLoopMax（闭环油泵给定上限）"
  Gain2/1 -> Bus Creator/5  "Nc_dem（控制目标转速）"
  Gain3/1 -> Bus Creator/6  "Ki（积分增益）"
  Gain4/1 -> Bus Creator/7  "Kp（比例增益）"
  Gain5/1 -> Bus Creator/8  "RotaSpeed_ErrorAllow（转速允许偏差）"
  Fault_Process/1(S_CloseLoop_Acclera tor_Out) -> Bus Creator/1, Scope1/1  "CloseLoop_Acclerator（闭环油泵给定）"
  CtrlLaw/1(S_CloseLoop_Acclerator) -> Fault_Process/3(S_CloseLoop_Acclerator)
  Switch/1 -> Bus Creator/9  "SWO_BleedAir（引气阀使能）"
  Bus Selector2/1 -> Fault_Process/2(S_Acclerator_Last), CtrlLaw/1(S_Acclerator_Last)  "<Accelerator（油泵给定控制量）>"
  [Nc_Filter] -> DaYu5000/1
  [S_SPM] -> Fault_Process/4(SPM)
  dth = T0-288.1/1 -> Switch/3
  dth = T0-288.6/1 -> Switch/1
  DaYu5000/1 -> Switch/2

== system turbo_controller/CLM/ControlOut_Manage ==
  note: 把当前模式的候选值合成统一执行总线
      |
      | 前面的Origin、Start、ClpControl、Manual、Stop分别算出了候选控制。本层接收这些结果和当前控
      | 制模式，不让五套候选同时驱动硬件。
      |
      | Accelerator_Manage负责油泵：按模式选出给定，闭环和手动分别受各自上下限约束；若复位恢复工作
      | 标志成立，采用恢复油泵值覆盖普通选择。
      | SWO_Manage负责主副阀、电机、点火与引气等字段：根据模式执行对应动作分支，再用Merge合成唯一
      | 结果。
      |
      | 最后Bus Creator按固定字段组成S_Servo_Out，包含油泵给定、各执行机构周期/开启计数/使能，以及
      | 点火等开关要求。ServoCtrlFlag记录油泵究竟来自正常分支还是上下限分支，供诊断使用。
      |
      | 输出交根层ControlOut整理端口，再由BoardOutput把周期计数变成电平、把给定变成串口帧。本模块
      | 完成的是控制量仲裁，尚未执行实际GPIO/UART动作。
  S_CtrlMode : Inport
      settings: AttributesFormatString=S_CtrlMode（控制模式）
  S_FAM : Inport  Port=2
      settings: AttributesFormatString=S_FAM（故障标志总线）
  S_Origin : Inport  Port=3
      settings: AttributesFormatString=S_Origin（原位）
  S_Start : Inport  Port=4
      settings: AttributesFormatString=S_Start（地面起动）
  S_CloseLoop : Inport  Port=5
      settings: AttributesFormatString=S_CloseLoop（闭合回路）
  S_Manual : Inport  Port=6
      settings: AttributesFormatString=S_Manual（手动）
  S_Stop_Accelerator : Inport  Port=7
      settings: AttributesFormatString=S_Stop_Accelerator（停车油门）
  S_SPM : Inport  Port=8
      settings: AttributesFormatString=S_SPM（通信及传感器信息总线）
  Accelerator_Manage : Subsystem  Description=|
      | 油泵给定最终从哪一路选择
      | 
      | 输入同时带有当前控制模式及五种模式的候选油泵值。ServoCtrlOut先按模式选择：原位取Vin_Origin，起动取Vin_Start，停车取Vin_Stop；闭环与手动则在各自最小/最大给定内限制候选值。
      | 
      | 例如闭环候选9000而上限8000，输出8000，并把ServoCtrlFlag置为闭环上限分支；正常处于范围内时保留候选值。这个标志用于告诉后面“为什么给了这个值”。
      | 
      | 图外LogicSelection3再看Flag_ECUReset_work：有效时采用恢复记录中的ECUReset_Acclerator，否则采用ServoCtrlOut的Vout。两层选择顺序不同，恢复支路是在模式选择之后。
      | 
      | 输出一路是给定值，另一路是选择标志，随后组成执行总线。当前上层恢复许可接false，不能因这里保留了恢复选择接口就认定实机一定使用了恢复数据。
      settings: AttributesFormatString=Accelerator_Manage（油门管理）
  Bus Creator : BusCreator  Inputs=13
      settings: AttributesFormatString=Bus Creator（总线创建器）
  Bus Selector1 : BusSelector  OutputSignals=Accelerator（油泵给定控制量）
      settings: AttributesFormatString=Bus Selector1（总线选择器1）
  Bus Selector2 : BusSelector  OutputSignals=Accelerator（油泵给定控制量）
      settings: AttributesFormatString=Bus Selector2（总线选择器2）
  Bus Selector3 : BusSelector  OutputSignals=Start_Accelerator（地面起动油泵给定）
      settings: AttributesFormatString=Bus Selector3（总线选择器3）
  Bus Selector4 : BusSelector  OutputSignals="CloseLoop_Acclerator（闭环油泵给定）,Close  LoopMin（闭环油泵给定下限）,CloseLoopMax（闭环油泵给定上限）"
      settings: AttributesFormatString=Bus Selector4（总线选择器4）
  Bus Selector5 : BusSelector  OutputSignals=Manual_Accelerator（手动油泵给定）,ManualAcc_Min（手动油泵给定下限）,ManualAcc_Max（手动油泵给定上限）
      settings: AttributesFormatString=Bus Selector5（总线选择器5）
  SWO_Manage : Subsystem  Description=|
      | 阀门电机等字段怎样随模式一起切换
      | 
      | 油泵给定已经在同级Accelerator_Manage单独处理；本层负责其余执行机构字段。输入有原位、起动、闭环、手动、停车各模式总线，以及当前控制模式。
      | 
      | Switch Case按模式只允许对应动作子系统运行，动作分支把那套周期、开启计数、使能、点火/引气等字段取出。Merge接收当前被执行分支的结果，不是把五个分支数值求和。
      | 
      | 这样可以保证例如切入停车时，阀门和电机字段来自停车候选，而不是仍取起动分支保存的旧值。非当前分支可能保留历史输出，不能将保持值当作当前有效要求。
      | 
      | 输出分别接入统一执行总线，再交ControlOut和BoardOutput。这里切换的是软件要求，2 ms阀门周期和1 ms点火节奏由板级输出层实现。
      settings: AttributesFormatString=SWO_Manage（点火及阀电机输出选择）
  S_Servo_Out : Outport
      settings: AttributesFormatString=S_Servo_Out（伺服输出）
  wires:
  S_Start/1 -> [S_Start]
  [S_Start] -> Bus Selector3/1
  S_CloseLoop/1 -> [S_CloseLoop]
  S_Manual/1 -> [S_Manual]
  Bus Creator/1 -> S_Servo_Out/1
  [S_Start] -> SWO_Manage/2(S_Start)
  S_CtrlMode/1 -> [S_CtrlMode]
  [S_CtrlMode] -> SWO_Manage/1(S_CtrlMode)
  Bus Selector3/1 -> Accelerator_Manage/4(S_Start_Accelerator)  "<Start_Accelerator（地面起动油泵给定）>"
  Bus Selector4/1 -> Accelerator_Manage/5(S_CloseLoop_Accelerator)  "<CloseLoop_Acclerator（闭环油泵给定）>"
  Bus Selector4/2 -> Accelerator_Manage/6(S_CloseLoop_CloseLoopMin)  "<Close  LoopMin（闭环油泵给定下限）>"
  Bus Selector4/3 -> Accelerator_Manage/7(S_CloseLoop_CloseLoopMax)  "<CloseLoopMax（闭环油泵给定上限）>"
  Bus Selector2/1 -> Accelerator_Manage/8(S_Stop_Accelerator)  "<Accelerator（油泵给定控制量）>"
  Bus Selector5/1 -> Accelerator_Manage/9(S_Manual_Accelerator)  "<Manual_Accelerator（手动油泵给定）>"
  Bus Selector5/2 -> Accelerator_Manage/10(S_ManualAccMin)  "<ManualAcc_Min（手动油泵给定下限）>"
  Bus Selector5/3 -> Accelerator_Manage/11(S_ManualAccMax)  "<ManualAcc_Max（手动油泵给定上限）>"
  Accelerator_Manage/2(S_Acclerator) -> Bus Creator/13  "Accelerator（油泵给定控制量）"
  Accelerator_Manage/1(S_ServoCtrlFlag) -> Bus Creator/12  "ServoCtrlFlag（执行控制状态标志）"
  [S_CtrlMode] -> Accelerator_Manage/2(S_CtrlMode)
  S_FAM/1 -> Accelerator_Manage/1(S_FAM)
  S_SPM/1 -> Accelerator_Manage/12(S_SPM)
  S_Origin/1 -> [S_Origin]
  [S_Origin] -> SWO_Manage/3(S_Origin)
  [S_Stop] -> SWO_Manage/4(S_Stop)
  [S_Origin] -> Bus Selector1/1
  Bus Selector1/1 -> Accelerator_Manage/3(S_Origin_Accelerator)  "<Accelerator（油泵给定控制量）>"
  S_Stop_Accelerator/1 -> [S_Stop]
  SWO_Manage/6(S_Motor_Open) -> Bus Creator/6  "Motor_Open（起动电机开通计数）"
  SWO_Manage/5(S_Motor_Cycle) -> Bus Creator/5  "Motor_Cycle（起动电机周期计数）"
  SWO_Manage/4(S_Eblast_Open) -> Bus Creator/4  "Eblast_Open（副油阀开通计数）"
  SWO_Manage/3(S_Eblast_Cycle) -> Bus Creator/3  "Eblast_Cycle（副油阀周期计数）"
  SWO_Manage/2(S_EValve_Open) -> Bus Creator/2  "EValve_Open（主油阀开通计数）"
  SWO_Manage/1(S_EValve_Cycle) -> Bus Creator/1  "EValve_Cycle（主油阀周期计数）"
  SWO_Manage/7(S_EValve_Enable) -> Bus Creator/7  "EValve_Enable（主油阀使能）"
  SWO_Manage/8(S_Eblast_Enable) -> Bus Creator/8  "Eblast_Enable（副油阀使能）"
  SWO_Manage/9(S_Motor_Enable) -> Bus Creator/9  "Motor_Enable（起动电机使能）"
  SWO_Manage/10(S_SWO_Firework) -> Bus Creator/10  "SWO_Firework（点火器使能）"
  [S_Stop] -> Bus Selector2/1
  [S_Manual] -> SWO_Manage/5(S_Manual)
  [S_Manual] -> Bus Selector5/1
  [S_CloseLoop] -> Bus Selector4/1
  [S_CloseLoop] -> SWO_Manage/6(S_CloseLoop)
  SWO_Manage/11(S_SWO_BleedAir) -> Bus Creator/11  "SWO_BleedAir（引气阀使能）"

== system turbo_controller/CLM/Manual ==
  note: 接收手动命令，分别保持各执行器的设定
      |
      | 只有运行模式选到Manual时，本分支的结果才参与最终输出。它把“新一帧有效、命令编号、命令数据
      | ”送往各执行器，避免一条泵命令同时改动阀门或点火器。
      |
      | 主油阀、副油阀分别设置开通比例；起动电机设置0～100的开通计数；点火器和引气阀把数据是否大于
      | 等于1变成开关。没有对应的新命令时，各通道保留自己的原设定，而不是全部清零。
      |
      | 油泵另有直接给定和加减两条途径，并受转速保护及范围限制。手动输出仍要经过ControlOut_Manage
      | 、ControlOut和板级输出，才形成UART字节或GPIO电平；手动设定并不等于硬件已执行成功。
  S_SPM : Inport
      settings: AttributesFormatString=S_SPM（通信及传感器信息总线）
  S_ServoOut_Last : Inport  Port=2
      settings: AttributesFormatString=S_ServoOut_Last（伺服输出上一周期）
  S_FAM : Inport  Port=3
      settings: AttributesFormatString=S_FAM（故障标志总线）
  Action Port : ActionPort  InitializeStates=reset  ActionPortLabel=case [ 3 ]:
      settings: AttributesFormatString=Action Port（动作端口）
  BleedAir_Control : Subsystem  Description=|
      | 手动设置引气阀，其他命令不改它
      | 
      | 同时满足“收到有效帧”和“命令为引气阀设置”时，读取Data6：Data6≥1输出开，Data6<1输出关。这里采用开关含义，不把Data6当成开度百分比。
      | 
      | 条件不满足时，从上一拍控制输出总线取回SWO_BleedAir，保持原来的引气阀状态。因此发送油泵命令不会顺带关闭引气阀。该结果随后进入统一开关量输出，由板级输出转换成硬件电平。
      settings: AttributesFormatString=BleedAir_Control（手动引气阀控制）
  Bus Creator1 : BusCreator  Inputs=14
      settings: AttributesFormatString=Bus Creator1（总线创建器1）
  Bus Selector : BusSelector  OutputSignals=COMM（通信信息总线）.Flag_rx_suc（接收成功标志）,COMM（通信信息总线）.Instr（控制指令）,COMM（通信信息总线）.COMM_Data6（接收指令第六数据项）
      settings: AttributesFormatString=Bus Selector（总线选择器）
  Bus Selector1 : BusSelector  OutputSignals=OverSpeed_Protect（超转保护）
      settings: AttributesFormatString=Bus Selector1（总线选择器1）
  Eblast_Control : Subsystem  Description=|
      | 把手动油阀开度换算为周期内的开通拍数
      | 
      | 先确认有效帧属于本阀的设置命令，再把命令数据Data6按百分数换算：开通计数 = Data6×30/100，并限制在0～30；周期固定为30。例：Data6=50得到开通15拍，Data6=100得到开通30拍。
      | 
      | 使能判断使用换算后的计数是否大于等于1，因此非常小的设定可能仍不使能阀门。没有本阀的新有效设置时，保持原设定。本处只生成周期、开通和使能三项，实际的2 ms输出节拍在板级输出中执行。
      | 
      | 若阀门周期30、开通15，在2 ms节拍下就是每60 ms开30 ms。不要把这里的“15”直接读成15 ms。
      settings: AttributesFormatString=Eblast_Control（手动副油阀控制）
  Firework_Control : Subsystem  Description=|
      | 手动设置点火器并记住上次选择
      | 
      | 先检查有效接收标志和点火器设置命令是否同时成立。成立时，Data6≥1表示开，Data6<1表示关；否则使用单拍延迟保存的旧值。输出又送回延迟块，因此一次有效命令会持续生效，直到下一次有效点火命令修改它。
      | 
      | 这里输出的是点火许可，最终的9拍开、1拍关节奏由BoardOutput中的点火时序模块产生。本处不直接生成GPIO脉冲。
      settings: AttributesFormatString=Firework_Control（手动点火器控制）
  ManualAcc_Min_Control : Subsystem  Description=|
      | 形成手动油泵给定，并限制直接设定的范围
      | 
      | 接收有效的手动直接设定命令时，把Data6限制在0～70，再乘以100，形成泵控制编码。例：Data6=35得到3500，Data6=90会先限制为70，输出7000。这是设备控制编码，不是油压或燃油流量。
      | 
      | 没有直接设定命令时，使用“手动加减”分支产生的保持值。选择器决定采用新设定还是保持路径，范围模块防止结果超出允许值。对外同时给出手动控制上下界0和15000，供后续统一输出处理。最终泵命令还会经过使能、限幅和字节打包，才发送到泵。
      settings: AttributesFormatString=ManualAcc_Min_Control（手动油门下限控制）
  ManualEValve_Control : Subsystem  Description=|
      | 把手动油阀开度换算为周期内的开通拍数
      | 
      | 先确认有效帧属于本阀的设置命令，再把命令数据Data6按百分数换算：开通计数 = Data6×30/100，并限制在0～30；周期固定为30。例：Data6=50得到开通15拍，Data6=100得到开通30拍。
      | 
      | 使能判断使用换算后的计数是否大于等于1，因此非常小的设定可能仍不使能阀门。没有本阀的新有效设置时，保持原设定。本处只生成周期、开通和使能三项，实际的2 ms输出节拍在板级输出中执行。
      | 
      | 若阀门周期30、开通15，在2 ms节拍下就是每60 ms开30 ms。不要把这里的“15”直接读成15 ms。
      settings: AttributesFormatString=ManualEValve_Control（手动主油阀控制）
  Motor_Control : Subsystem  Description=|
      | 把手动命令转换为起动电机开通设定
      | 
      | 只有有效帧且命令属于电机设置时才更新。Data6直接作为开通计数，限制为0～100；周期固定100。原数据达到1才设置电机使能，否则关闭。
      | 
      | 例如Data6=40表示100个节拍中开40拍，不表示40 rpm。未收到相应命令时使用延迟记住上次的周期、开通和使能。结果由输出管理与板级时序继续处理，本模块不读取电机实际转速，也不进行速度闭环。
      settings: AttributesFormatString=Motor_Control（手动起动电机控制）
  N1r_idle6 : Constant  Value=PG_CtrlMode_ManualAcc  OutDataTypeStr=uint8  SampleTime=-1
      settings: AttributesFormatString=N1r_idle6（一级转速归一化值慢车6）
  Signal Conversion : SignalConversion  OverrideOpt=off
      settings: AttributesFormatString=Signal Conversion（信号转换）
  S_CtrlMode_ManualAcc : Outport  InitialOutput=[0]
      settings: AttributesFormatString=S_CtrlMode_ManualAcc（控制模式手动油门）
  S_Manual : Outport  Port=2
      settings: AttributesFormatString=S_Manual（手动）
  wires:
  N1r_idle6/1 -> S_CtrlMode_ManualAcc/1
  S_SPM/1 -> Bus Selector/1
  Signal Conversion/1 -> S_Manual/1
  ManualAcc_Min_Control/1(S_ManualAcc) -> Bus Creator1/1  "Manual_Accelerator（手动油泵给定）"
  Bus Creator1/1 -> Signal Conversion/1
  ManualEValve_Control/1(S_EValve_Cycle) -> Bus Creator1/4  "EValve_Cycle（主油阀周期计数）"
  Eblast_Control/2(S_Eblast_Open) -> Bus Creator1/8  "Eblast_Open（副油阀开通计数）"
  Eblast_Control/1(S_Eblast_Cycle) -> Bus Creator1/7  "Eblast_Cycle（副油阀周期计数）"
  ManualEValve_Control/2(S_EValve_Open) -> Bus Creator1/5  "EValve_Open（主油阀开通计数）"
  ManualEValve_Control/3(S_EValve_Enable) -> Bus Creator1/6  "EValve_Enable（主油阀使能）"
  Motor_Control/3(S_Motor_Enable) -> Bus Creator1/12  "Motor_Enable（起动电机使能）"
  Motor_Control/1(S_Motor_Cycle) -> Bus Creator1/10  "Motor_Cycle（起动电机周期计数）"
  Firework_Control/1(S_SWO_Firework) -> Bus Creator1/13  "SWO_Firework（点火器使能）"
  Motor_Control/2(S_Motor_Open) -> Bus Creator1/11  "Motor_Open（起动电机开通计数）"
  Eblast_Control/3(S_Eblast_Enable) -> Bus Creator1/9  "Eblast_Enable（副油阀使能）"
  Bus Selector/1 -> BleedAir_Control/1(S_Flag_rs_suc), Firework_Control/1(S_Flag_rs_suc), Motor_Control/1(S_Flag_rs_suc), Eblast_Control/1(S_Flag_rs_suc), ManualEValve_Control/1(S_Flag_rs_suc), ManualAcc_Min_Control/1(S_Flag_rs_suc)  "<Flag_rx_suc（接收成功标志）>"
  Bus Selector/2 -> BleedAir_Control/2(S_Instr), Firework_Control/2(S_Instr), Motor_Control/2(S_Instr), Eblast_Control/2(S_Instr), ManualEValve_Control/2(S_Instr), ManualAcc_Min_Control/2(S_Instr)  "<Instr（控制指令）>"
  S_ServoOut_Last/1 -> BleedAir_Control/4(S_ServoOut_Last), ManualEValve_Control/4(S_ServoOut_Last), ManualAcc_Min_Control/3(S_ServoOut_Last)
  Bus Selector/3 -> BleedAir_Control/3(S_COMM_Data6), Firework_Control/3(S_COMM_Data6), Motor_Control/3(S_COMM_Data6), Eblast_Control/3(S_COMM_Data6), ManualEValve_Control/3(S_COMM_Data6), ManualAcc_Min_Control/4(S_COMM_Data6)  "<COMM_Data6（接收指令第六数据项）>"
  ManualAcc_Min_Control/3(S_ManualAcc_Max) -> Bus Creator1/3  "ManualAcc_Max（手动油泵给定上限）"
  ManualAcc_Min_Control/2(S_ManualAcc_Min) -> Bus Creator1/2  "ManualAcc_Min（手动油泵给定下限）"
  BleedAir_Control/1(S_SWO_BleedAirSet) -> Bus Creator1/14  "SWO_BleedAir（引气阀使能）"
  S_FAM/1 -> Bus Selector1/1
  Bus Selector1/1 -> ManualAcc_Min_Control/5(S_OverSpeed_Protect)  "<OverSpeed_Protect（超转保护）>"

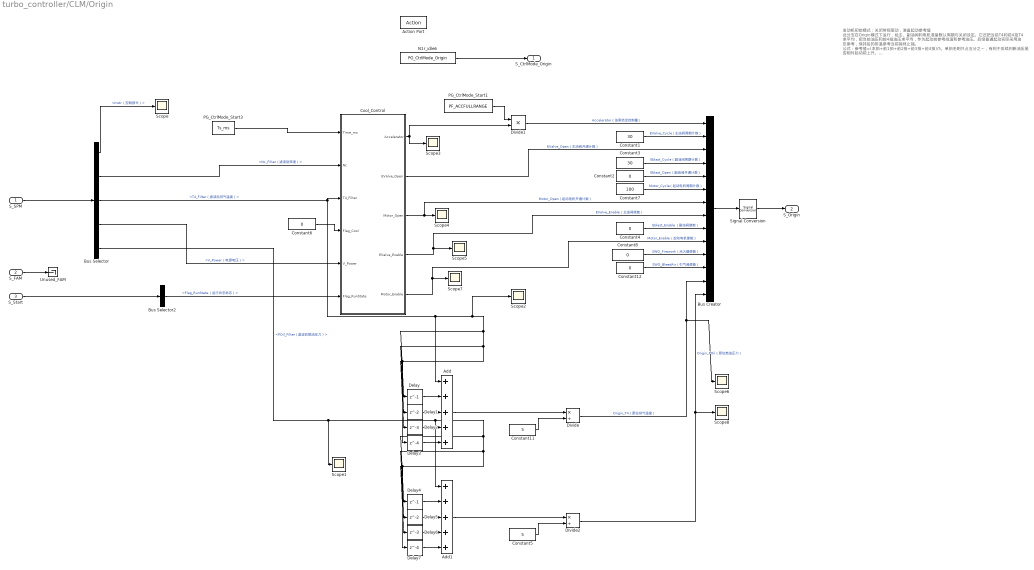
== system turbo_controller/CLM/Origin ==
  note: 发动机初始模式：关闭常规驱动，准备起动参考值
      |
      | 此分支在Origin模式下运行，给主、副油阀和电机准备默认周期与关闭设定。它还把当前T4和前4拍T4
      | 求平均，把当前油压和前4拍油压求平均，作为起动前参考排温和参考油压。后续普通起动实际采用油
      | 压参考，保持后的排温参考当前接终止端。
      |
      | 公式：参考值=(本拍+前1拍+前2拍+前3拍+前4拍)/5。单拍毛刺只占五分之一，有利于后续判断油压是
      | 否相对起动前上升。
      |
      | 内部保留Cool_Control冷却顺序，但当前接入它的Flag_Cool是常量0，正常连接下不会发起该冷却过程
      | 。不要仅因看到冷却控制图就认为初始模式一定会开电机吹冷。输出分别送模式选择和Start的参考值
      | 保持路径。
  S_SPM : Inport
      settings: AttributesFormatString=S_SPM（通信及传感器信息总线）
  S_FAM : Inport  Port=2
      settings: AttributesFormatString=S_FAM（故障标志总线）
  S_Start : Inport  Port=3
      settings: AttributesFormatString=S_Start（地面起动）
  Action Port : ActionPort  InitializeStates=reset  ActionPortLabel=case [ 0 ]:
      settings: AttributesFormatString=Action Port（动作端口）
  Add : Sum  Inputs=+++++
      settings: AttributesFormatString=Add（加法求和）
  Add1 : Sum  Inputs=+++++
      settings: AttributesFormatString=Add1（加法求和1）
  Bus Creator : BusCreator  Inputs=14
      settings: AttributesFormatString=Bus Creator（总线创建器）
  Bus Selector : BusSelector  OutputSignals=COMM（通信信息总线）.Instr（控制指令）,Sensor（传感器信息总线）.Nc_Filter（滤波后转速）,Sensor（传感器信息总线）.T4_Filter（滤波后排气温度）,COMM（通信信息总线）.V_Power（电源电压）,Sensor（传感器信息总线）.POil_Filter（滤波后燃油压力）
      settings: AttributesFormatString=Bus Selector（总线选择器）
  Bus Selector2 : BusSelector  OutputSignals=Flag_RunState（运行状态标志）
      settings: AttributesFormatString=Bus Selector2（总线选择器2）
  Constant1 : Constant  Value=30  OutDataTypeStr=uint16  SampleTime=-1
      settings: AttributesFormatString=Constant1（常量1）
  Constant11 : Constant  Value=5  OutDataTypeStr=single  SampleTime=-1
      settings: AttributesFormatString=Constant11（常量11）
  Constant12 : Constant  Value=0  OutDataTypeStr=uint8  SampleTime=-1
      settings: AttributesFormatString=Constant12（常量12）
  Constant2 : Constant  Value=0  OutDataTypeStr=uint16  SampleTime=-1
      settings: AttributesFormatString=Constant2（常量2）
  Constant3 : Constant  Value=30  OutDataTypeStr=uint16  SampleTime=-1
      settings: AttributesFormatString=Constant3（常量3）
  Constant4 : Constant  Value=0  OutDataTypeStr=uint8  SampleTime=-1
      settings: AttributesFormatString=Constant4（常量4）
  Constant5 : Constant  Value=5  OutDataTypeStr=single  SampleTime=-1
      settings: AttributesFormatString=Constant5（常量5）
  Constant6 : Constant  Value=0  OutDataTypeStr=boolean  SampleTime=-1
      settings: AttributesFormatString=Constant6（常量6）
  Constant7 : Constant  Value=100  OutDataTypeStr=uint16  SampleTime=-1
      settings: AttributesFormatString=Constant7（常量7）
  Constant8 : Constant  Value=0  OutDataTypeStr=uint8  SampleTime=-1
      settings: AttributesFormatString=Constant8（常量8）
  Cool_Control : Stateflow chart  Description=|  TreatAsAtomicUnit=on  RTWFcnName=Timmer  RTWFileName=MCM_Timmer
      | 保留的停车冷却时序；当前请求端固定为0
      | 
      | 本图用于收到冷却请求后按阶段控制起动电机、油泵及主油阀。Flag_Cool为假会撤销冷却过程、清总计数和完成标志；当前父系统把该输入接为常量0，因此这些主动冷却阶段目前不会投入。
      | 
      | 若以后接入有效请求，图内有低转速检查和40、60等电机开通设定，并以30 s、40 s、50 s、70 s等计时点推进。供油支路按0.1×28/V_Power补偿供电变化；T4<110参与结束供油判断，120 s作为总流程退出限制。
      | 
      | 时间比较采用毫秒/Time_ms换成调用次数，而不是每个计数代表1 s。V_Power来自父级选定信号，不能仅凭名称认定是ADC供电通道。此图保留算法，但实际是否运行由请求连接决定。
      settings: AttributesFormatString=Cool_Control（冷却控制）  RTWFcnNameOpts=Use subsystem name  RTWFileNameOpts=User specified
  Delay : Delay  DelayLength=1
      settings: AttributesFormatString=Delay（延迟）
  Delay1 : Delay
      settings: AttributesFormatString=Delay1（延迟1）
  Delay2 : Delay  DelayLength=3
      settings: AttributesFormatString=Delay2（延迟2）
  Delay3 : Delay  DelayLength=4
      settings: AttributesFormatString=Delay3（延迟3）
  Delay4 : Delay  DelayLength=1
      settings: AttributesFormatString=Delay4（延迟4）
  Delay5 : Delay
      settings: AttributesFormatString=Delay5（延迟5）
  Delay6 : Delay  DelayLength=3
      settings: AttributesFormatString=Delay6（延迟6）
  Delay7 : Delay  DelayLength=4
      settings: AttributesFormatString=Delay7（延迟7）
  Divide : Product  Inputs=*/
      settings: AttributesFormatString=Divide（除法）
  Divide1 : Product  Inputs=**
      settings: AttributesFormatString=Divide1（除法1）
  Divide2 : Product  Inputs=*/
      settings: AttributesFormatString=Divide2（除法2）
  N1r_idle6 : Constant  Value=PG_CtrlMode_Origin  OutDataTypeStr=uint8  SampleTime=-1
      settings: AttributesFormatString=N1r_idle6（一级转速归一化值慢车6）
  PG_CtrlMode_Start1 : Constant  Value=PF_ACCFULLRANGE  OutDataTypeStr=single  SampleTime=-1
      settings: AttributesFormatString=PG_CtrlMode_Start1（起动1）
  PG_CtrlMode_Start3 : Constant  Value=Ts_ms  SampleTime=-1
      settings: AttributesFormatString=PG_CtrlMode_Start3（起动3）
  Scope{,1..8} (9 alike) : Scope
      Scope settings: AttributesFormatString=Scope（示波器）  ActiveDisplayYMinimum=-0.125  ActiveDisplayYMaximum=1.125
      Scope1 settings: AttributesFormatString=Scope1（示波器1）  ActiveDisplayYMinimum=80.17242  ActiveDisplayYMaximum=657.75848  DataLoggingVariableName=ScopeData2
      Scope2 settings: AttributesFormatString=Scope2（示波器2）  ActiveDisplayYMinimum=-0.38306  ActiveDisplayYMaximum=3.44752  DataLoggingVariableName=ScopeData7
      Scope3 settings: AttributesFormatString=Scope3（示波器3）  ActiveDisplayYMinimum=-1  ActiveDisplayYMaximum=1  DataLoggingVariableName=ScopeData3
      Scope4 settings: AttributesFormatString=Scope4（示波器4）  ActiveDisplayYMinimum=-1  ActiveDisplayYMaximum=1  DataLoggingVariableName=ScopeData4
      Scope5 settings: AttributesFormatString=Scope5（示波器5）  ActiveDisplayYMinimum=-0.125  ActiveDisplayYMaximum=1.125  DataLoggingVariableName=ScopeData3
      Scope6 settings: AttributesFormatString=Scope6（示波器6）  ActiveDisplayYMinimum=-0.31469  ActiveDisplayYMaximum=2.8322  DataLoggingVariableName=ScopeData8
      Scope7 settings: AttributesFormatString=Scope7（示波器7）  ActiveDisplayYMinimum=-0.125  ActiveDisplayYMaximum=1.125  DataLoggingVariableName=ScopeData4
      Scope8 settings: AttributesFormatString=Scope8（示波器8）  ActiveDisplayYMinimum=-43.9655  ActiveDisplayYMaximum=671.55159  DataLoggingVariableName=ScopeData2
  Signal Conversion : SignalConversion  OverrideOpt=off
      settings: AttributesFormatString=Signal Conversion（信号转换）
  Unused_FAM : Terminator
  S_CtrlMode_Origin : Outport  InitialOutput=[0]
      settings: AttributesFormatString=S_CtrlMode_Origin（控制模式原位）
  S_Origin : Outport  Port=2  OutputWhenDisabled=reset  InitialOutput=[0]
      settings: AttributesFormatString=S_Origin（原位）
  wires:
  Constant4/1 -> Bus Creator/9  "Eblast_Enable（副油阀使能）"
  Cool_Control/1(Accelerator) -> Divide1/2, Scope3/1
  PG_CtrlMode_Start1/1 -> Divide1/1
  Bus Selector/2 -> Cool_Control/2(Nc)  "<Nc_Filter（滤波后转速）>"
  PG_CtrlMode_Start3/1 -> Cool_Control/1(Time_ms)
  Bus Selector/1 -> Scope/1  "<Instr（控制指令）>"
  Constant12/1 -> Bus Creator/12  "SWO_BleedAir（引气阀使能）"
  Constant11/1 -> Divide/2
  Add/1 -> Divide/1
  Divide/1 -> Bus Creator/13, Scope6/1  "Origin_T4（原位排气温度）"
  Delay1/1 -> Add/3
  Delay2/1 -> Add/4
  Delay3/1 -> Add/5
  Delay/1 -> Add/2
  Bus Selector/3 -> Delay/1, Delay1/1, Delay2/1, Delay3/1, Scope2/1, Add/1, Cool_Control/3(T4_Filter)  "<T4_Filter（滤波后排气温度）>"
  S_SPM/1 -> Bus Selector/1
  Cool_Control/3(Motor_Open) -> Bus Creator/7, Scope4/1  "Motor_Open（起动电机开通计数）"
  Constant8/1 -> Bus Creator/11  "SWO_Firework（点火器使能）"
  Constant7/1 -> Bus Creator/6  "Motor_Cycle（起动电机周期计数）"
  Cool_Control/5(Motor_Enable) -> Bus Creator/10, Scope7/1  "Motor_Enable（起动电机使能）"
  Cool_Control/4(EValve_Enable) -> Bus Creator/8, Scope5/1  "EValve_Enable（主油阀使能）"
  Cool_Control/2(EValve_Open) -> Bus Creator/3  "EValve_Open（主油阀开通计数）"
  Constant3/1 -> Bus Creator/4  "Eblast_Cycle（副油阀周期计数）"
  Constant2/1 -> Bus Creator/5  "Eblast_Open（副油阀开通计数）"
  Constant1/1 -> Bus Creator/2  "EValve_Cycle（主油阀周期计数）"
  Signal Conversion/1 -> S_Origin/1
  Bus Creator/1 -> Signal Conversion/1
  N1r_idle6/1 -> S_CtrlMode_Origin/1
  Divide1/1 -> Bus Creator/1  "Accelerator（油泵给定控制量）"
  Constant6/1 -> Cool_Control/4(Flag_Cool)
  Bus Selector/4 -> Cool_Control/5(V_Power)  "<V_Power（电源电压）>"
  S_Start/1 -> Bus Selector2/1
  Bus Selector2/1 -> Cool_Control/6(Flag_RunState)  "<Flag_RunState（运行状态标志）>"
  Constant5/1 -> Divide2/2
  Add1/1 -> Divide2/1
  Divide2/1 -> Scope8/1, Bus Creator/14  "Origin_POil（原位燃油压力）"
  Delay5/1 -> Add1/3
  Delay6/1 -> Add1/4
  Delay7/1 -> Add1/5
  Delay4/1 -> Add1/2
  Bus Selector/5 -> Delay7/1, Delay6/1, Delay5/1, Delay4/1, Add1/1, Scope1/1  "<POil_Filter（滤波后燃油压力）>"
  S_FAM/1 -> Unused_FAM/1
